simulink model "day2_pwm_open_loop"  (R2026a)
settings: Solver=VariableStepAuto
undefined symbols (not defined in the file): b, J, Ke, Kt, L, R, rad_to_rpm, T_load, V_supply
settings Model: Creator=DELL  LastModifiedBy=DELL

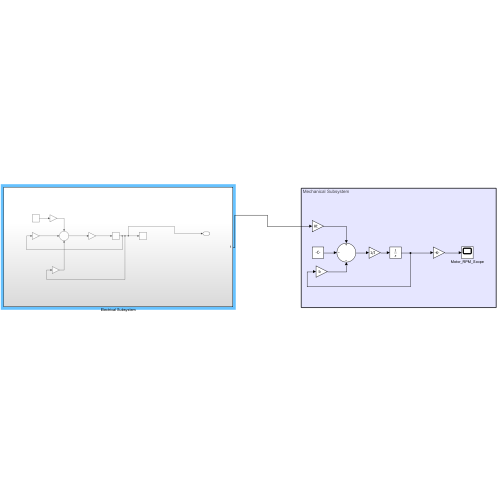
[thumbnail: Simulink's stored preview of the top-level diagram]
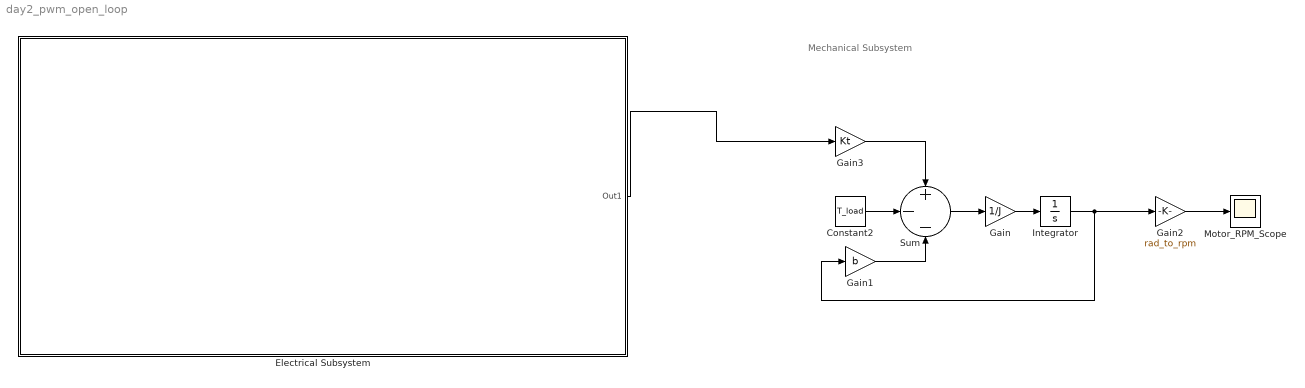
== system day2_pwm_open_loop ==
  note: Mechanical Subsystem
  Constant2 : Constant  Value=T_load
  Electrical Subsystem : Subsystem
  Gain : Gain  Gain=1/J
  Gain1 : Gain  Gain=b
  Gain2 : Gain  Gain=rad_to_rpm
  Gain3 : Gain  Gain=Kt
  Integrator : Integrator
  Motor_RPM_Scope : Scope
      settings: ActiveDisplayYMinimum=-5469.5785327149169  ActiveDisplayYMaximum=41734.903297781719
  Sum : Sum  Inputs=+--
  wires:
  Gain3/1 -> Sum/1
  Gain/1 -> Integrator/1
  Sum/1 -> Gain/1
  Constant2/1 -> Sum/2
  Gain2/1 -> Motor_RPM_Scope/1
  Gain1/1 -> Sum/3
  Integrator/1 -> Gain1/1, Gain2/1
  Electrical Subsystem/1(Out1) -> Gain3/1

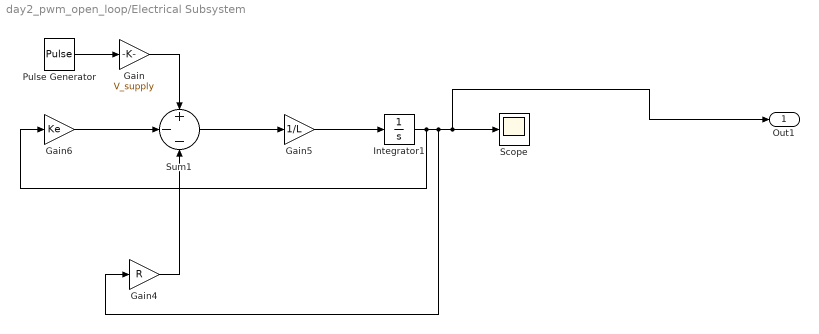
== system day2_pwm_open_loop/Electrical Subsystem ==
  Gain : Gain  Gain=V_supply
  Gain4 : Gain  Gain=R
  Gain5 : Gain  Gain=1/L
  Gain6 : Gain  Gain=Ke
  Integrator1 : Integrator
  Pulse Generator : DiscretePulseGenerator  PulseType=Time based  Period=10  PulseWidth=5
  Scope : Scope
      settings: ActiveDisplayYMinimum=-0.046366756718675572  ActiveDisplayYMaximum=4.9531791851211349
  Sum1 : Sum  Inputs=+--
  Out1 : Outport
  wires:
  Integrator1/1 -> Gain6/1, Gain4/1, Out1/1, Scope/1
  Sum1/1 -> Gain5/1
  Gain/1 -> Sum1/1
  Gain5/1 -> Integrator1/1
  Gain6/1 -> Sum1/2
  Gain4/1 -> Sum1/3
  Pulse Generator/1 -> Gain/1
